simulink model "kundur_sync"  (R2023b)
settings: Solver=ode23tb  StartTime=0.0  StopTime=200  MaxStep=1/60  RelTol=1e-3
InitFcn:
  | SolarInverter_Params();
values from neighbouring files (symbols this model uses):
  Fnom = 60    [SolarInverter_Params.m]
  Pnom = 900e6    (= 900000000)    [SolarInverter_Params.m]
  reec_dbd1 = -0.1    [SolarInverter_Params.m]
  reec_dbd2 = 0.1    [SolarInverter_Params.m]
  reec_dPmax = 0.1    [SolarInverter_Params.m]
  reec_dPmin = -0.1    [SolarInverter_Params.m]
  reec_Imax = 1    [SolarInverter_Params.m]
  reec_Iqhl = 1.0    (= 1)    [SolarInverter_Params.m]
  reec_Iqll = -0.4    [SolarInverter_Params.m]
  reec_Kqi = 0.0    (= 0)    [SolarInverter_Params.m]
  reec_Kqp = 0    [SolarInverter_Params.m]
  reec_Kvi = 0.0    (= 0)    [SolarInverter_Params.m]
  reec_Kvp = 0.1    [SolarInverter_Params.m]
  reec_Pmax = 1.0    (= 1)    [SolarInverter_Params.m]
  reec_Pmin = 0    [SolarInverter_Params.m]
  reec_Qmax = 0.435    [SolarInverter_Params.m]
  reec_Qmin = -0.435    [SolarInverter_Params.m]
  reec_Tiq = 0.02    [SolarInverter_Params.m]
  reec_Tp = 0.02    [SolarInverter_Params.m]
  reec_Tpord = 0.1    [SolarInverter_Params.m]
  reec_Trv = 0.01    [SolarInverter_Params.m]
  reec_Vdip = 0.9    [SolarInverter_Params.m]
  reec_Vmax = 1.10    (= 1.1)    [SolarInverter_Params.m]
  reec_Vmin = 0.9    [SolarInverter_Params.m]
  reec_Vup = 1.15    [SolarInverter_Params.m]
  regc_Brkpt = 0.9    [SolarInverter_Params.m]
  regc_Iolim = -1.2    [SolarInverter_Params.m]
  regc_Iqrmax = 999.9    [SolarInverter_Params.m]
  regc_Iqrmin = -999.9    [SolarInverter_Params.m]
  regc_Ivpnt0 = 0.4    [SolarInverter_Params.m]
  regc_Ivpnt1 = 0.8    [SolarInverter_Params.m]
  regc_Khv = 0.0    (= 0)    [SolarInverter_Params.m]
  regc_Lvpl1 = 1.0    (= 1)    [SolarInverter_Params.m]
  regc_Lvplsw = 0    [SolarInverter_Params.m]
  regc_rrpwr = 10    [SolarInverter_Params.m]
  regc_Tfltr = 0.02    [SolarInverter_Params.m]
  regc_Tg = 0.1    [SolarInverter_Params.m]
  regc_Volim = 1.1    [SolarInverter_Params.m]
  regc_Zerox = 0.5    [SolarInverter_Params.m]
  repc_db1 = 0    [SolarInverter_Params.m]
  repc_Ddn = 20    [SolarInverter_Params.m]
  repc_Dup = 0    [SolarInverter_Params.m]
  repc_emax = 999    [SolarInverter_Params.m]
  repc_emin = -999    [SolarInverter_Params.m]
  repc_fdbd1 = 0.01*0    (= 0)    [SolarInverter_Params.m]
  repc_fdbd2 = -0.01*0    (= 0)    [SolarInverter_Params.m]
  repc_femax = 999    [SolarInverter_Params.m]
  repc_femin = -999    [SolarInverter_Params.m]
  repc_Kc = 0.05    [SolarInverter_Params.m]
  repc_Ki = 1.8    [SolarInverter_Params.m]
  repc_Kig = 0.5    [SolarInverter_Params.m]
  repc_Kp = 0.6    [SolarInverter_Params.m]
  repc_Kpg = 0.1    [SolarInverter_Params.m]
  repc_Pmax = 1    [SolarInverter_Params.m]
  repc_Pmin = 0    [SolarInverter_Params.m]
  repc_Qmax = 0.435    [SolarInverter_Params.m]
  repc_Qmin = -0.435    [SolarInverter_Params.m]
  repc_Rc = 0    [SolarInverter_Params.m]
  repc_Tfltr = 0.02    [SolarInverter_Params.m]
  repc_Tft = 0.5    [SolarInverter_Params.m]
  repc_Tfv = 0.8    [SolarInverter_Params.m]
  repc_Tlag = 0.2    [SolarInverter_Params.m]
  repc_Tp = 0.25    [SolarInverter_Params.m]
  repc_Vfrz = 0.7    [SolarInverter_Params.m]
  repc_Xc = 0    [SolarInverter_Params.m]
  Vnom = 230e3    (= 230000)    [SolarInverter_Params.m]
undefined symbols (not defined in the file or in its folder): D1, Delta, gcbh, j, k_fault, k_pulse, sps_rtmsupport
libraries: powerlib_extras x24, simulink x13, spsLoadFlowBusLib x12, spsThreePhaseVIMeasurementLib x11, spsThreePhasePISectionLineLib x8, spsThreePhaseTransformerTwoWindingsLib x5, spsThreePhaseParallelRLCLoadLib x4, spsSynchronousMachinepuStandardLib x4, spsExcitationSystemLib x4, spsSteamTurbineandGovernorLib x4, spsGenericPowerSystemStabilizerLib x4, spsControlledCurrentSourceLib x2
(part 2 of 3)

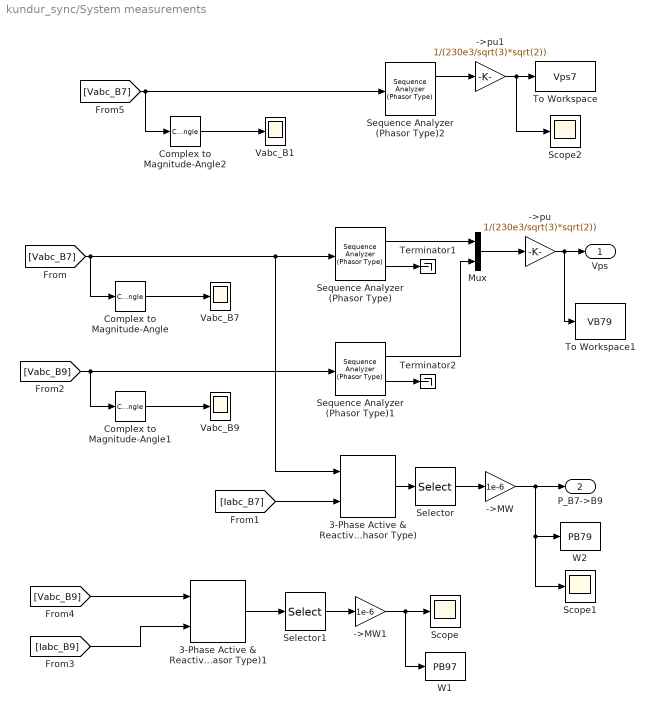
== system kundur_sync/System measurements ==
  ->MW : Gain  Gain=1e-6  SaturateOnIntegerOverflow=on  OutDataTypeStr=Inherit: Same as input  ParamDataTypeStr=Inherit: Same as input
  ->MW1 : Gain  Gain=1e-6  SaturateOnIntegerOverflow=on  OutDataTypeStr=Inherit: Same as input  ParamDataTypeStr=Inherit: Same as input
  ->pu : Gain  Gain=1/(230e3/sqrt(3)*sqrt(2))  SaturateOnIntegerOverflow=on  OutDataTypeStr=Inherit: Same as input  ParamDataTypeStr=Inherit: Same as input
  ->pu1 : Gain  Gain=1/(230e3/sqrt(3)*sqrt(2))  SaturateOnIntegerOverflow=on  OutDataTypeStr=Inherit: Same as input  ParamDataTypeStr=Inherit: Same as input
  3-Phase Active & Reactive Power (Phasor Type) : powerlib_extras/Phasor Library/3-Phase Active & Reactive Power (Phasor Type)
  3-Phase Active & Reactive Power (Phasor Type)1 : powerlib_extras/Phasor Library/3-Phase Active & Reactive Power (Phasor Type)
  Complex to Magnitude-Angle : ComplexToMagnitudeAngle  Output=Magnitude
  Complex to Magnitude-Angle1 : ComplexToMagnitudeAngle  Output=Magnitude
  Complex to Magnitude-Angle2 : ComplexToMagnitudeAngle  Output=Magnitude
  Mux : Mux  Inputs=2
  Scope : Scope
  Scope1 : Scope
  Scope2 : Scope
  Selector : Selector  InputPortWidth=2  IndexOptions=Index vector (dialog)  Indices=1  OutputSizes=1
  Selector1 : Selector  InputPortWidth=2  IndexOptions=Index vector (dialog)  Indices=1  OutputSizes=1
  Sequence Analyzer (Phasor Type) : powerlib_extras/Phasor Library/Sequence Analyzer (Phasor Type)  seq=Positive
  Sequence Analyzer (Phasor Type)1 : powerlib_extras/Phasor Library/Sequence Analyzer (Phasor Type)  seq=Positive
  Sequence Analyzer (Phasor Type)2 : powerlib_extras/Phasor Library/Sequence Analyzer (Phasor Type)  seq=Positive
  Terminator1 : Terminator
  Terminator2 : Terminator
  To Workspace : ToWorkspace  VariableName=Vps7  SampleTime=1/60
  To Workspace1 : ToWorkspace  VariableName=VB79  SampleTime=1/60
  Vabc_B1 : Scope
  Vabc_B7 : Scope
  Vabc_B9 : Scope
  W1 : ToWorkspace  VariableName=PB97  SampleTime=1/60
  W2 : ToWorkspace  VariableName=PB79  SampleTime=1/60
  Vps : Outport  VectorParamsAs1DForOutWhenUnconnected=off
  P_B7->B9 : Outport  Port=2  VectorParamsAs1DForOutWhenUnconnected=off
  wires:
  Mux/1 -> ->pu/1
  ->MW/1 -> P_B7->B9/1, Scope1/1, W2/1
  Complex to Magnitude-Angle/1 -> Vabc_B7/1
  Sequence Analyzer (Phasor Type)/1 -> Mux/1
  Selector/1 -> ->MW/1
  Sequence Analyzer (Phasor Type)/2 -> Terminator1/1
  ->pu/1 -> To Workspace1/1, Vps/1
  [Iabc_B9] -> 3-Phase Active & Reactive Power (Phasor Type)1/2
  [Iabc_B7] -> 3-Phase Active & Reactive Power (Phasor Type)/2
  3-Phase Active & Reactive Power (Phasor Type)/1 -> Selector/1
  Sequence Analyzer (Phasor Type)1/1 -> Mux/2
  Complex to Magnitude-Angle1/1 -> Vabc_B9/1
  [Vabc_B9] -> Sequence Analyzer (Phasor Type)1/1, Complex to Magnitude-Angle1/1
  [Vabc_B7] -> Sequence Analyzer (Phasor Type)/1, 3-Phase Active & Reactive Power (Phasor Type)/1, Complex to Magnitude-Angle/1
  Sequence Analyzer (Phasor Type)1/2 -> Terminator2/1
  [Vabc_B9] -> 3-Phase Active & Reactive Power (Phasor Type)1/1
  ->MW1/1 -> Scope/1, W1/1
  3-Phase Active & Reactive Power (Phasor Type)1/1 -> Selector1/1
  Selector1/1 -> ->MW1/1
  Complex to Magnitude-Angle2/1 -> Vabc_B1/1
  [Vabc_B7] -> Sequence Analyzer (Phasor Type)2/1, Complex to Magnitude-Angle2/1
  Sequence Analyzer (Phasor Type)2/1 -> ->pu1/1
  ->pu1/1 -> Scope2/1, To Workspace/1

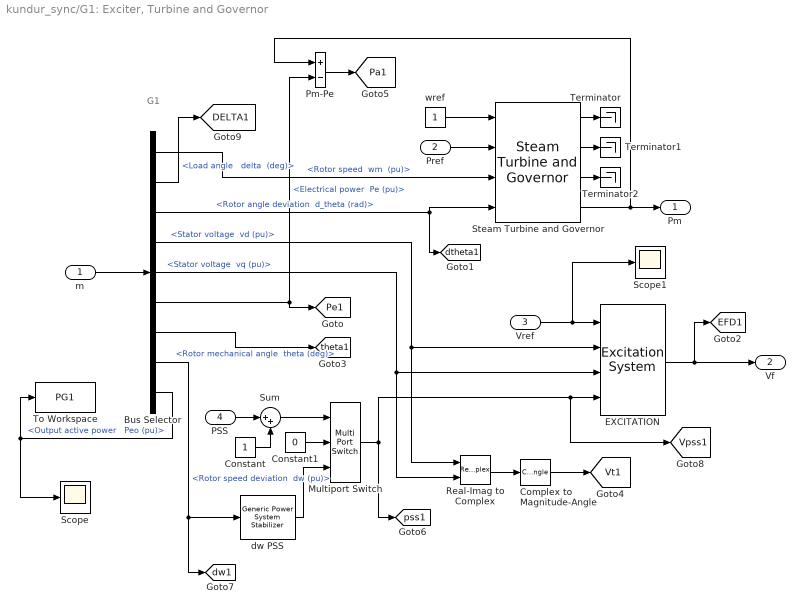
== system kundur_sync/G1: Exciter, Turbine and Governor ==
  note: G1
  m : Inport
  Pref : Inport  Port=2
  Vref : Inport  Port=3
  PSS : Inport  Port=4
  Bus Selector : BusSelector  OutputSignals="Mechanical.Rotor speed  wm  (pu),Load angle   delta  (deg),Mechanical.Rotor angle deviation  d_theta (rad),dq0 components.Stator voltage  vd (pu),dq0 components.Stator voltage  vq (pu),Mechanical.Electrical power  Pe (pu),Mechanical.Rotor mechanical angle  theta (deg),Mechanical.Rotor speed deviation  dw (pu),Output active power   Peo (pu)"
  Complex to Magnitude-Angle : ComplexToMagnitudeAngle  Output=Magnitude
  Constant : Constant
  Constant1 : Constant  Value=0
  EXCITATION : spsExcitationSystemLib/Excitation System  tr=20e-3  reg=[ 200, 0.001 ]  exc=[ 1, 0 ]  tgr=[ 0, 0 ]  damp=[ 0, 0 ]  sat=[ 0, 0 ]  lim=[ 0 , 12.3, 0 ]  v0=[1.03 1.9356]
  Multiport Switch : MultiPortSwitch  Inputs=2  SaturateOnIntegerOverflow=off  InputSameDT=off
  Pm-Pe : Sum  Inputs=+-
  Real-Imag to Complex : RealImagToComplex
  Scope : Scope
  Scope1 : Scope
  Sum : Sum  Inputs=|++
  Terminator : Terminator
  Terminator1 : Terminator
  Terminator2 : Terminator
  To Workspace : ToWorkspace  VariableName=PG1  SampleTime=1/60
  Steam Turbine and Governor : spsSteamTurbineandGovernorLib/Steam Turbine and Governor  gentype=Tandem-compound (single mass)  reg1="[ 1  0.05    0 ]"  reg2="[ 0.001  0.15 ]"  reg3="[ -0.1  0.1  0  4.496]"  N=3600  turb1="[ 0  10  3.3  0.5 ]"  turb2="[ 0   0.36   0.36  0.28 ]"  HA="[  1.5498   0.24894  0  0 ]"  KA="[  83.47  42.702  0  0 ]"  DA="[  0.3104  0.05  0  0 ]*8"  ini1=0.7793  ini2=[2.7247e-008,-120.13]
      settings: LibrarySourceBlock=|
      | sps_lib/Electrical Machines/Synchronous Machine Control/Steam Turbine
      | and Governor
  dw PSS : spsGenericPowerSystemStabilizerLib/Generic Power System Stabilizer  Tsensor=15e-3  K=30  Twashout=10  Tleadlag1=[50e-3 20e-3]  Tleadlag2=[3 5.4]  VSlimits=[-0.15 0.15]  Vinit=0  Plot_On=off  MagdB_On=on  FreqRange=logspace(-2,2,500)
      settings: LibrarySourceBlock=|
      | sps_lib/Electrical Machines/Synchronous Machine Control/Generic
      | Power System Stabilizer
  wref : Constant
  Pm : Outport  VectorParamsAs1DForOutWhenUnconnected=off
  Vf : Outport  Port=2  VectorParamsAs1DForOutWhenUnconnected=off
  tag scope: DELTA1=global, EFD1=global, Pa1=global, Pe1=global, Vpss1=global, Vt1=global, dtheta1=global, dw1=global, pss1=global, theta1=global
  wires:
  m/1 -> Bus Selector/1
  Steam Turbine and Governor/4 -> Pm/1, Pm-Pe/1
  Bus Selector/1 -> Steam Turbine and Governor/3  "<Rotor speed  wm  (pu)>"
  Bus Selector/3 -> Steam Turbine and Governor/4, [dtheta1]  "<Rotor angle deviation  d_theta (rad)>"
  Bus Selector/4 -> Real-Imag to Complex/1, EXCITATION/2  "<Stator voltage  vd (pu)>"
  Bus Selector/5 -> Real-Imag to Complex/2, EXCITATION/3  "<Stator voltage  vq (pu)>"
  wref/1 -> Steam Turbine and Governor/1
  Pref/1 -> Steam Turbine and Governor/2
  Steam Turbine and Governor/1 -> Terminator/1
  Steam Turbine and Governor/2 -> Terminator1/1
  Steam Turbine and Governor/3 -> Terminator2/1
  Bus Selector/6 -> Pm-Pe/2, [Pe1]  "<Electrical power  Pe (pu)>"
  Bus Selector/7 -> [theta1]  "<Rotor mechanical angle  theta (deg)>"
  Real-Imag to Complex/1 -> Complex to Magnitude-Angle/1
  Complex to Magnitude-Angle/1 -> [Vt1]
  Bus Selector/8 -> [dw1], dw PSS/1  "<Rotor speed deviation  dw (pu)>"
  Sum/1 -> Multiport Switch/1
  PSS/1 -> Sum/1
  Constant/1 -> Sum/2
  Constant1/1 -> Multiport Switch/2
  dw PSS/1 -> Multiport Switch/3
  Multiport Switch/1 -> [Vpss1], EXCITATION/4, [pss1]
  Pm-Pe/1 -> [Pa1]
  Bus Selector/9 -> Scope/1, To Workspace/1  "<Output active power   Peo (pu)>"
  EXCITATION/1 -> [EFD1], Vf/1
  Vref/1 -> Scope1/1, EXCITATION/1
  Bus Selector/2 -> [DELTA1]  "<Load angle   delta  (deg)>"

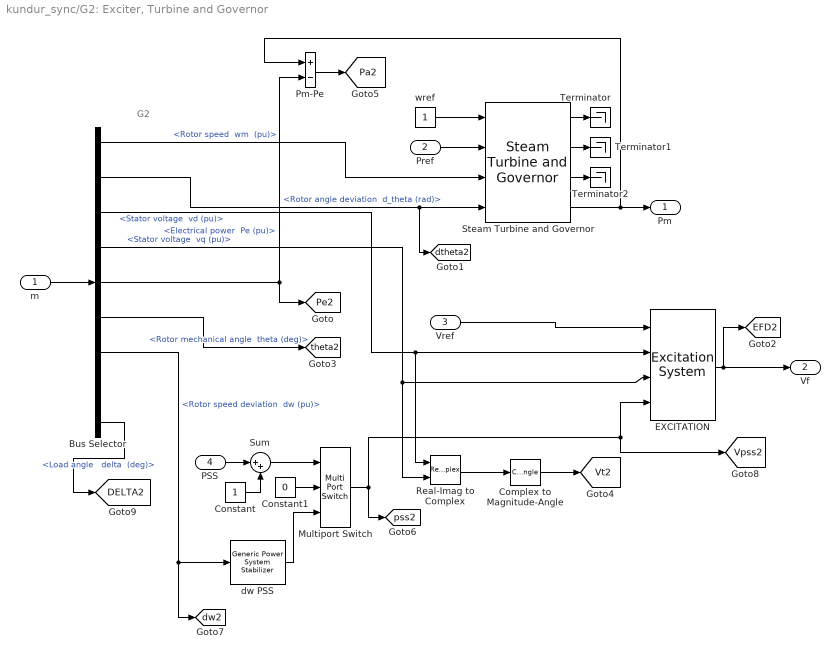
== system kundur_sync/G2: Exciter, Turbine and Governor ==
  note: G2
  m : Inport
  Pref : Inport  Port=2
  Vref : Inport  Port=3
  PSS : Inport  Port=4
  Bus Selector : BusSelector  OutputSignals="Mechanical.Rotor speed  wm  (pu),Mechanical.Rotor angle deviation  d_theta (rad),dq0 components.Stator voltage  vd (pu),dq0 components.Stator voltage  vq (pu),Mechanical.Electrical power  Pe (pu),Mechanical.Rotor mechanical angle  theta (deg),Mechanical.Rotor speed deviation  dw (pu),dq0 components.Field current  ifd (pu),Load angle   delta  (deg)"
  Complex to Magnitude-Angle : ComplexToMagnitudeAngle  Output=Magnitude
  Constant : Constant
  Constant1 : Constant  Value=0
  EXCITATION : spsExcitationSystemLib/Excitation System  tr=20e-3  reg=[ 200, 0.001 ]  exc=[ 1, 0 ]  tgr=[ 0, 0 ]  damp=[ 0, 0 ]  sat=[ 0, 0 ]  lim=[ 0 , 12.3, 0 ]  v0=[1.01 2.0029]
  Multiport Switch : MultiPortSwitch  Inputs=2  SaturateOnIntegerOverflow=off  InputSameDT=off
  Pm-Pe : Sum  Inputs=+-
  Real-Imag to Complex : RealImagToComplex
  Sum : Sum  Inputs=|++
  Terminator : Terminator
  Terminator1 : Terminator
  Terminator2 : Terminator
  Steam Turbine and Governor : spsSteamTurbineandGovernorLib/Steam Turbine and Governor  gentype=Tandem-compound (single mass)  reg1="[ 1  0.05    0 ]"  reg2="[ 0.001  0.15 ]"  reg3="[ -0.1  0.1  0  4.496]"  N=3600  turb1="[ 0  10   3.3   0.5   ]"  turb2="[ 0   0.36   0.36  0.28 ]"  HA="[  1.5498   0.24894  0  0 ]"  KA="[  83.47  42.702  0  0 ]"  DA="[  0.3104  0.05  0  0 ]*8"  ini1=0.77941  ini2=[2.7247e-008,-120.13]
      settings: LibrarySourceBlock=|
      | sps_lib/Electrical Machines/Synchronous Machine Control/Steam Turbine
      | and Governor
  dw PSS : spsGenericPowerSystemStabilizerLib/Generic Power System Stabilizer  Tsensor=15e-3  K=30  Twashout=10  Tleadlag1=[50e-3 20e-3]  Tleadlag2=[3 5.4]  VSlimits=[-0.15 0.15]  Vinit=0  Plot_On=off  MagdB_On=on  FreqRange=logspace(-2,2,500)
      settings: LibrarySourceBlock=|
      | sps_lib/Electrical Machines/Synchronous Machine Control/Generic
      | Power System Stabilizer
  wref : Constant
  Pm : Outport  VectorParamsAs1DForOutWhenUnconnected=off
  Vf : Outport  Port=2  VectorParamsAs1DForOutWhenUnconnected=off
  tag scope: DELTA2=global, EFD2=global, Pa2=global, Pe2=global, Vpss2=global, Vt2=global, dtheta2=global, dw2=global, pss2=global, theta2=global
  wires:
  m/1 -> Bus Selector/1
  EXCITATION/1 -> Vf/1, [EFD2]
  Steam Turbine and Governor/4 -> Pm/1, Pm-Pe/1
  Bus Selector/1 -> Steam Turbine and Governor/3  "<Rotor speed  wm  (pu)>"
  Bus Selector/2 -> Steam Turbine and Governor/4, [dtheta2]  "<Rotor angle deviation  d_theta (rad)>"
  Bus Selector/3 -> Real-Imag to Complex/1, EXCITATION/2  "<Stator voltage  vd (pu)>"
  Bus Selector/4 -> EXCITATION/3, Real-Imag to Complex/2  "<Stator voltage  vq (pu)>"
  wref/1 -> Steam Turbine and Governor/1
  Pref/1 -> Steam Turbine and Governor/2
  Steam Turbine and Governor/1 -> Terminator/1
  Steam Turbine and Governor/2 -> Terminator1/1
  Steam Turbine and Governor/3 -> Terminator2/1
  Vref/1 -> EXCITATION/1
  Bus Selector/5 -> [Pe2], Pm-Pe/2  "<Electrical power  Pe (pu)>"
  Bus Selector/6 -> [theta2]  "<Rotor mechanical angle  theta (deg)>"
  Real-Imag to Complex/1 -> Complex to Magnitude-Angle/1
  Complex to Magnitude-Angle/1 -> [Vt2]
  Sum/1 -> Multiport Switch/1
  PSS/1 -> Sum/1
  Constant/1 -> Sum/2
  Constant1/1 -> Multiport Switch/2
  dw PSS/1 -> Multiport Switch/3
  Multiport Switch/1 -> [Vpss2], EXCITATION/4, [pss2]
  Pm-Pe/1 -> [Pa2]
  Bus Selector/7 -> [dw2], dw PSS/1  "<Rotor speed deviation  dw (pu)>"
  Bus Selector/9 -> [DELTA2]  "<Load angle   delta  (deg)>"

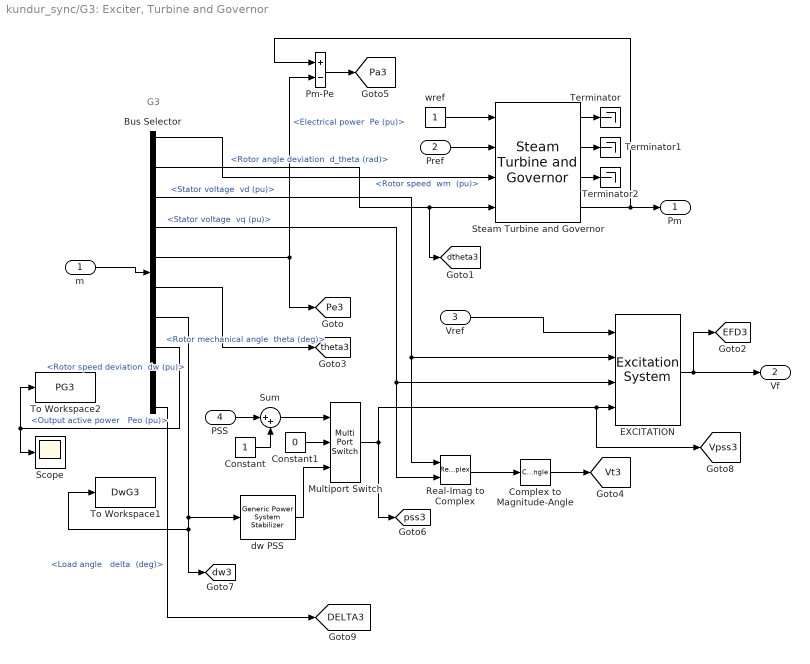
== system kundur_sync/G3: Exciter, Turbine and Governor ==
  note: G3
  m : Inport
  Pref : Inport  Port=2
  Vref : Inport  Port=3
  PSS : Inport  Port=4
  Bus Selector : BusSelector  OutputSignals="Mechanical.Rotor speed  wm  (pu),Mechanical.Rotor angle deviation  d_theta (rad),dq0 components.Stator voltage  vd (pu),dq0 components.Stator voltage  vq (pu),Mechanical.Electrical power  Pe (pu),Mechanical.Rotor mechanical angle  theta (deg),Mechanical.Rotor speed deviation  dw (pu),Output active power   Peo (pu),dq0 components.Field current  ifd (pu),Load angle   delta  (deg)"
  Complex to Magnitude-Angle : ComplexToMagnitudeAngle  Output=Magnitude
  Constant : Constant
  Constant1 : Constant  Value=0
  EXCITATION : spsExcitationSystemLib/Excitation System  tr=20e-3  reg=[ 200, 0.001 ]  exc=[ 1, 0 ]  tgr=[ 0, 0 ]  damp=[ 0, 0 ]  sat=[ 0, 0 ]  lim=[ 0 , 12.3, 0 ]  v0=[1.03 1.9474]
  Multiport Switch : MultiPortSwitch  Inputs=2  SaturateOnIntegerOverflow=off  InputSameDT=off
  Pm-Pe : Sum  Inputs=+-
  Real-Imag to Complex : RealImagToComplex
  Scope : Scope
  Sum : Sum  Inputs=|++
  Terminator : Terminator
  Terminator1 : Terminator
  Terminator2 : Terminator
  To Workspace1 : ToWorkspace  VariableName=DwG3  SampleTime=1/60
  To Workspace2 : ToWorkspace  VariableName=PG3  SampleTime=1/60
  Steam Turbine and Governor : spsSteamTurbineandGovernorLib/Steam Turbine and Governor  gentype=Tandem-compound (single mass)  reg1="[ 1  0.05    0 ]"  reg2="[ 0.001  0.15 ]"  reg3="[ -0.1  0.1  0  4.496]"  N=3600  turb1="[ 0  10   3.3   0.5   ]"  turb2="[ 0   0.36   0.36  0.28 ]"  HA="[  1.5498   0.24894  0  0 ]"  KA="[  83.47  42.702  0  0 ]"  DA="[  0.3104  0.05  0  0 ]*8"  ini1=0.80012  ini2=[2.7247e-008,-120.13]
      settings: LibrarySourceBlock=|
      | sps_lib/Electrical Machines/Synchronous Machine Control/Steam Turbine
      | and Governor
  dw PSS : spsGenericPowerSystemStabilizerLib/Generic Power System Stabilizer  Tsensor=15e-3  K=30  Twashout=10  Tleadlag1=[50e-3 20e-3]  Tleadlag2=[3 5.4]  VSlimits=[-0.15 0.15]  Vinit=0  Plot_On=off  MagdB_On=on  FreqRange=logspace(-2,2,500)
      settings: LibrarySourceBlock=|
      | sps_lib/Electrical Machines/Synchronous Machine Control/Generic
      | Power System Stabilizer
  wref : Constant
  Pm : Outport  VectorParamsAs1DForOutWhenUnconnected=off
  Vf : Outport  Port=2  VectorParamsAs1DForOutWhenUnconnected=off
  tag scope: DELTA3=global, EFD3=global, Pa3=global, Pe3=global, Vpss3=global, Vt3=global, dtheta3=global, dw3=global, pss3=global, theta3=global
  wires:
  m/1 -> Bus Selector/1
  EXCITATION/1 -> Vf/1, [EFD3]
  Steam Turbine and Governor/4 -> Pm/1, Pm-Pe/1
  Bus Selector/1 -> Steam Turbine and Governor/3  "<Rotor speed  wm  (pu)>"
  Bus Selector/2 -> Steam Turbine and Governor/4, [dtheta3]  "<Rotor angle deviation  d_theta (rad)>"
  Bus Selector/3 -> EXCITATION/2, Real-Imag to Complex/1  "<Stator voltage  vd (pu)>"
  Bus Selector/4 -> Real-Imag to Complex/2, EXCITATION/3  "<Stator voltage  vq (pu)>"
  wref/1 -> Steam Turbine and Governor/1
  Pref/1 -> Steam Turbine and Governor/2
  Steam Turbine and Governor/1 -> Terminator/1
  Steam Turbine and Governor/2 -> Terminator1/1
  Steam Turbine and Governor/3 -> Terminator2/1
  Vref/1 -> EXCITATION/1
  Bus Selector/5 -> [Pe3], Pm-Pe/2  "<Electrical power  Pe (pu)>"
  Bus Selector/6 -> [theta3]  "<Rotor mechanical angle  theta (deg)>"
  Real-Imag to Complex/1 -> Complex to Magnitude-Angle/1
  Complex to Magnitude-Angle/1 -> [Vt3]
  Sum/1 -> Multiport Switch/1
  PSS/1 -> Sum/1
  Constant/1 -> Sum/2
  Constant1/1 -> Multiport Switch/2
  dw PSS/1 -> Multiport Switch/3
  Multiport Switch/1 -> [Vpss3], EXCITATION/4, [pss3]
  Pm-Pe/1 -> [Pa3]
  Bus Selector/7 -> To Workspace1/1, [dw3], dw PSS/1  "<Rotor speed deviation  dw (pu)>"
  Bus Selector/8 -> Scope/1, To Workspace2/1  "<Output active power   Peo (pu)>"
  Bus Selector/10 -> [DELTA3]  "<Load angle   delta  (deg)>"

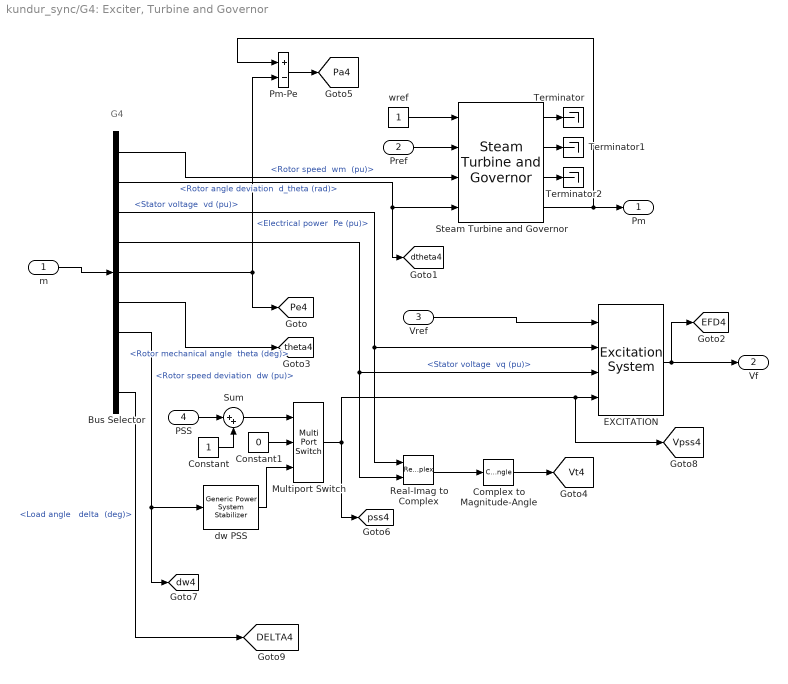
== system kundur_sync/G4: Exciter, Turbine and Governor ==
  note: G4
  m : Inport
  Pref : Inport  Port=2
  Vref : Inport  Port=3
  PSS : Inport  Port=4
  Bus Selector : BusSelector  OutputSignals="Mechanical.Rotor speed  wm  (pu),Mechanical.Rotor angle deviation  d_theta (rad),dq0 components.Stator voltage  vd (pu),dq0 components.Stator voltage  vq (pu),Mechanical.Electrical power  Pe (pu),Mechanical.Rotor mechanical angle  theta (deg),Mechanical.Rotor speed deviation  dw (pu),dq0 components.Field current  ifd (pu),Load angle   delta  (deg)"
  Complex to Magnitude-Angle : ComplexToMagnitudeAngle  Output=Magnitude
  Constant : Constant
  Constant1 : Constant  Value=0
  EXCITATION : spsExcitationSystemLib/Excitation System  tr=20e-3  reg=[ 200, 0.001 ]  exc=[ 1, 0 ]  tgr=[ 0, 0 ]  damp=[ 0, 0 ]  sat=[ 0, 0 ]  lim=[ 0 , 12.3, 0 ]  v0=[1.01 1.9533]
  Multiport Switch : MultiPortSwitch  Inputs=2  SaturateOnIntegerOverflow=off  InputSameDT=off
  Pm-Pe : Sum  Inputs=+-
  Real-Imag to Complex : RealImagToComplex
  Sum : Sum  Inputs=|++
  Terminator : Terminator
  Terminator1 : Terminator
  Terminator2 : Terminator
  Steam Turbine and Governor : spsSteamTurbineandGovernorLib/Steam Turbine and Governor  gentype=Tandem-compound (single mass)  reg1="[ 1  0.05    0 ]"  reg2="[ 0.001  0.15 ]"  reg3="[ -0.1  0.1  0  4.496]"  N=3600  turb1="[ 0  10   3.3   0.5   ]"  turb2="[ 0   0.36   0.36  0.28 ]"  HA="[  1.5498   0.24894  0  0 ]"  KA="[  83.47  42.702  0  0 ]"  DA="[  0.3104  0.05  0  0 ]*8"  ini1=0.77936  ini2=[2.7247e-008,-120.13]
      settings: LibrarySourceBlock=|
      | sps_lib/Electrical Machines/Synchronous Machine Control/Steam Turbine
      | and Governor
  dw PSS : spsGenericPowerSystemStabilizerLib/Generic Power System Stabilizer  Tsensor=15e-3  K=30  Twashout=10  Tleadlag1=[50e-3 20e-3]  Tleadlag2=[3 5.4]  VSlimits=[-0.15 0.15]  Vinit=0  Plot_On=off  MagdB_On=on  FreqRange=logspace(-2,2,500)
      settings: LibrarySourceBlock=|
      | sps_lib/Electrical Machines/Synchronous Machine Control/Generic
      | Power System Stabilizer
  wref : Constant
  Pm : Outport  VectorParamsAs1DForOutWhenUnconnected=off
  Vf : Outport  Port=2  VectorParamsAs1DForOutWhenUnconnected=off
  tag scope: DELTA4=global, EFD4=global, Pa4=global, Pe4=global, Vpss4=global, Vt4=global, dtheta4=global, dw4=global, pss4=global, theta4=global
  wires:
  m/1 -> Bus Selector/1
  EXCITATION/1 -> [EFD4], Vf/1
  Steam Turbine and Governor/4 -> Pm/1, Pm-Pe/1
  Bus Selector/1 -> Steam Turbine and Governor/3  "<Rotor speed  wm  (pu)>"
  Bus Selector/2 -> Steam Turbine and Governor/4, [dtheta4]  "<Rotor angle deviation  d_theta (rad)>"
  Bus Selector/3 -> EXCITATION/2, Real-Imag to Complex/1  "<Stator voltage  vd (pu)>"
  Bus Selector/4 -> EXCITATION/3, Real-Imag to Complex/2  "<Stator voltage  vq (pu)>"
  wref/1 -> Steam Turbine and Governor/1
  Pref/1 -> Steam Turbine and Governor/2
  Steam Turbine and Governor/1 -> Terminator/1
  Steam Turbine and Governor/2 -> Terminator1/1
  Steam Turbine and Governor/3 -> Terminator2/1
  Vref/1 -> EXCITATION/1
  Bus Selector/5 -> [Pe4], Pm-Pe/2  "<Electrical power  Pe (pu)>"
  Bus Selector/6 -> [theta4]  "<Rotor mechanical angle  theta (deg)>"
  Real-Imag to Complex/1 -> Complex to Magnitude-Angle/1
  Complex to Magnitude-Angle/1 -> [Vt4]
  Sum/1 -> Multiport Switch/1
  PSS/1 -> Sum/1
  Constant/1 -> Sum/2
  Constant1/1 -> Multiport Switch/2
  dw PSS/1 -> Multiport Switch/3
  Multiport Switch/1 -> [Vpss4], EXCITATION/4, [pss4]
  Pm-Pe/1 -> [Pa4]
  Bus Selector/7 -> [dw4], dw PSS/1  "<Rotor speed deviation  dw (pu)>"
  Bus Selector/9 -> [DELTA4]  "<Load angle   delta  (deg)>"

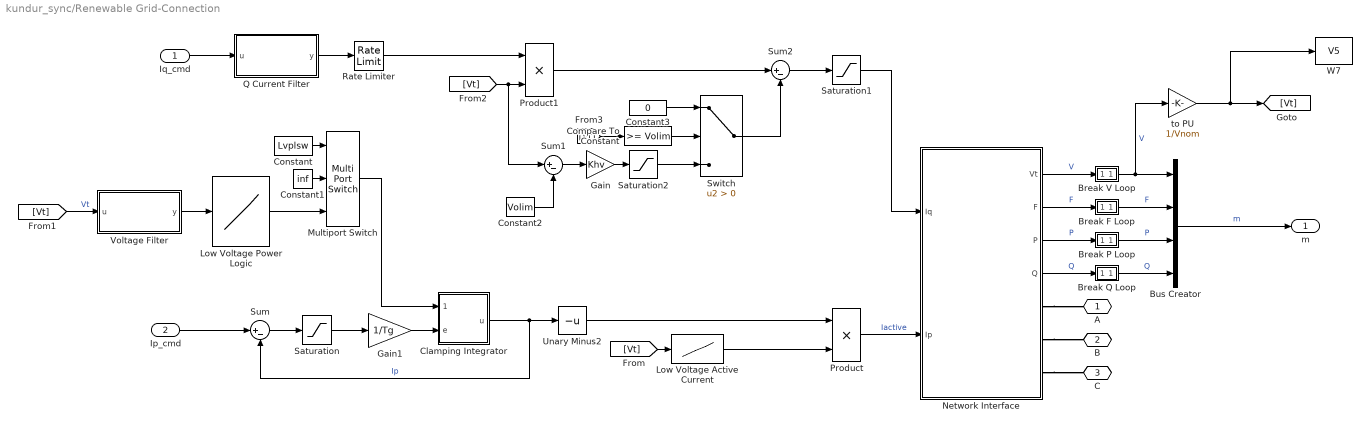
== system kundur_sync/Renewable Grid-Connection ==
  Iq_cmd : Inport
  Ip_cmd : Inport  Port=2
  Break F Loop : Subsystem  mask{tau=0.001, toPU=Fnom}
      mask prompts: toPU "Convert to PU"
  Break P Loop : Subsystem  mask{tau=0.001, toPU=Pnom}
      mask prompts: toPU "Convert to PU"
  Break Q Loop : Subsystem  mask{tau=0.001, toPU=Pnom}
      mask prompts: toPU "Convert to PU"
  Break V Loop : Subsystem  mask{tau=0.001, toPU=Vnom}
      mask prompts: toPU "Convert to PU"
  Bus Creator : BusCreator  Inputs=4
  Clamping Integrator : Subsystem
  Compare To Constant : simulink/Logic and Bit Operations/Compare To Constant  relop=>=  const=Volim  OutDataTypeStr=boolean
  Constant : Constant  Value=Lvplsw
  Constant1 : Constant  Value=inf
  Constant2 : Constant  Value=Volim
  Constant3 : Constant  Value=0
  Gain : Gain  Gain=Khv
  Gain1 : Gain  Gain=1/Tg
  Low Voltage Active Current : Lookup_n-D  NumberOfTableDimensions=1  BreakpointsForDimension1=[0 Ivpnt0 Ivpnt1 Ivpnt1*1.5]  Table=[0 0 1 1]  InternalRulePriority=Speed  RndMeth=Simplest
  Low Voltage Power Logic : Lookup_n-D  NumberOfTableDimensions=1  BreakpointsForDimension1=[0 Zerox Brkpt Brkpt*1.01 Brkpt*1.5]  Table=[0 0 Lvpl1 Lvpl1*5 Lvpl1*5]  InternalRulePriority=Speed  RndMeth=Simplest
  Multiport Switch : MultiPortSwitch  DataPortOrder=Zero-based contiguous  Inputs=2  zeroidx=on  SaturateOnIntegerOverflow=off  InputSameDT=off
  Network Interface : Subsystem
  Product : Product
  Product1 : Product
  Q Current Filter : Subsystem  mask{k=1, tau=Tg, vmax=Iqrmax, vmin=Iqrmin}
      mask Display: fprintf('1\n------------\n(1 + s Tg)');
  Rate Limiter : RateLimiter  RisingSlewLimit=Iqrmax  FallingSlewLimit=Iqrmin  SampleTimeMode=inherited
  Saturation : Saturate  UpperLimit=rrpwr  LowerLimit=-inf
  Saturation1 : Saturate  UpperLimit=inf  LowerLimit=Iolim
  Saturation2 : Saturate  UpperLimit=inf  LowerLimit=0
  Sum : Sum  Inputs=|+-
  Sum1 : Sum  Inputs=|+-
  Sum2 : Sum  Inputs=|+-
  Switch : Switch  Criteria=u2 > Threshold  SaturateOnIntegerOverflow=off  InputSameDT=off
  Unary Minus2 : UnaryMinus
  Voltage Filter : Subsystem  mask{k=1, tau=Tfltr, vmax=inf, vmin=-inf}
      mask Display: fprintf('1\n------------\n(1 + s Tfltr)');
  W7 : ToWorkspace  VariableName=V5  SampleTime=1/60
  to PU : Gain  Gain=1/Vnom
  A : PMIOPort  Side=Right
  B : PMIOPort  Port=2  Side=Right
  C : PMIOPort  Port=3  Side=Right
  m : Outport  VectorParamsAs1DForOutWhenUnconnected=off
  wires:
  [Vt] -> Voltage Filter/1(u)  "Vt"
  Q Current Filter/1(y) -> Rate Limiter/1
  Network Interface/4(Q) -> Break Q Loop/1(u)  "Q"
  Constant3/1 -> Switch/1
  Network Interface/1(Vt) -> Break V Loop/1(u)  "V"
  Iq_cmd/1 -> Q Current Filter/1(u)
  Gain/1 -> Saturation2/1
  Network Interface/3(P) -> Break P Loop/1(u)  "P"
  Voltage Filter/1(y) -> Low Voltage Power Logic/1
  Constant1/1 -> Multiport Switch/2
  Sum/1 -> Saturation/1
  Constant/1 -> Multiport Switch/1
  Product/1 -> Network Interface/2(Ip)  "Iactive"
  Low Voltage Active Current/1 -> Product/2
  Multiport Switch/1 -> Clamping Integrator/1(LVMax)
  Clamping Integrator/1(u) -> Sum/2, Unary Minus2/1  "Ip"
  Gain1/1 -> Clamping Integrator/2(e)
  [Vt] -> Compare To Constant/1
  Saturation/1 -> Gain1/1
  [Vt] -> Low Voltage Active Current/1
  Constant2/1 -> Sum1/2
  Saturation1/1 -> Network Interface/1(Iq)
  Product1/1 -> Sum2/1
  Sum1/1 -> Gain/1
  Rate Limiter/1 -> Product1/1
  Saturation2/1 -> Switch/3
  [Vt] -> Sum1/1, Product1/2
  Low Voltage Power Logic/1 -> Multiport Switch/3
  Compare To Constant/1 -> Switch/2
  Switch/1 -> Sum2/2
  Bus Creator/1 -> m/1  "m"
  Sum2/1 -> Saturation1/1
  Ip_cmd/1 -> Sum/1
  Network Interface/2(F) -> Break F Loop/1(u)  "F"
  Unary Minus2/1 -> Product/1
  to PU/1 -> W7/1, [Vt]
  Break V Loop/1(y) -> to PU/1, Bus Creator/1  "V"
  Break F Loop/1(y) -> Bus Creator/2  "F"
  Break P Loop/1(y) -> Bus Creator/3  "P"
  Break Q Loop/1(y) -> Bus Creator/4  "Q"
  connections:
  Network Interface/RConn3 -- C/RConn1
  Network Interface/RConn1 -- A/RConn1
  Network Interface/RConn2 -- B/RConn1

== system kundur_sync/Selection ==
  In1 : Inport
  Bus Selector : BusSelector  OutputSignals=V,F,P,Q
  Mux : Mux  Inputs=2
  Mux1 : Mux  Inputs=2
  Mux2 : Mux  Inputs=2
  P to PU : Gain  Gain=1/Pnom
  Q to PU : Gain  Gain=1/Pnom
  V to PU : Gain  Gain=1/Vnom
  Out1 : Outport
  <F> : Outport  Port=2
  Out3 : Outport  Port=3
  Out4 : Outport  Port=4
  wires:
  Bus Selector/4 -> Q to PU/1  "<Q>"
  Bus Selector/3 -> P to PU/1  "<P>"
  V to PU/1 -> Mux2/1
  Bus Selector/1 -> V to PU/1  "<V>"
  [Vref] -> Mux2/2
  Q to PU/1 -> Mux1/1
  P to PU/1 -> Mux/1
  [Qref] -> Mux1/2
  [Pref] -> Mux/2
  Bus Selector/2 -> <F>/1  "<F>"
  Mux/1 -> Out3/1
  Mux2/1 -> Out1/1
  Mux1/1 -> Out4/1
  In1/1 -> Bus Selector/1

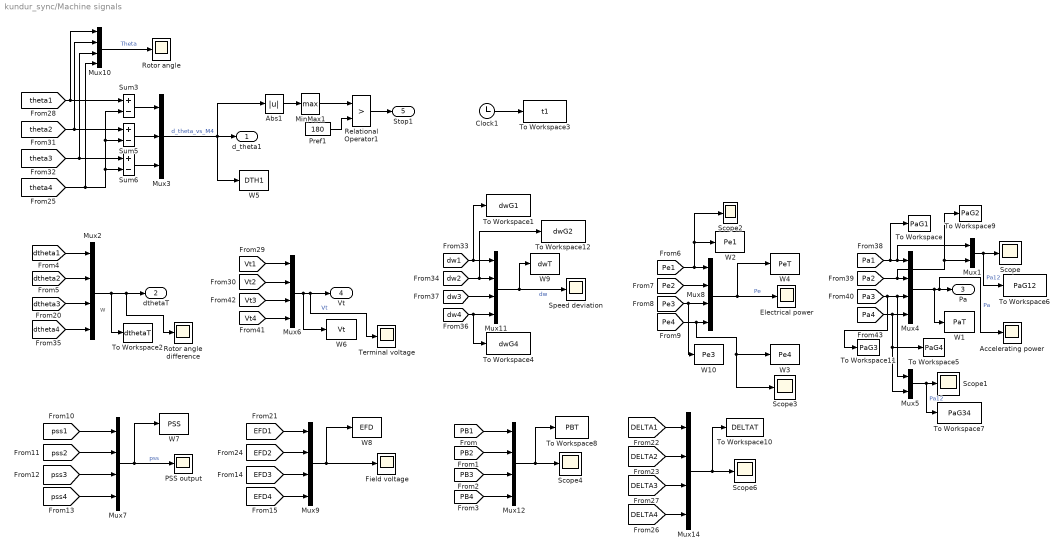
== system kundur_sync/Machine signals ==
  note: w
  Abs1 : Abs
  Clock1 : Clock
  Speed deviation : Scope
  Rotor angle difference : Scope
  MinMax1 : MinMax  Function=max  InputSameDT=on  SaturateOnIntegerOverflow=on
  Mux1 : Mux  Inputs=2
  Mux{2,4,6..12,14} (10 alike) : Mux
  Mux3 : Mux  Inputs=3
  Mux5 : Mux  Inputs=2
  Electrical power : Scope
  Accelerating power : Scope
  Pref1 : Constant  Value=180
  Relational Operator1 : RelationalOperator  Operator=>
  Scope{,1..4,6} (6 alike) : Scope
  PSS output : Scope
  Sum3 : Sum  Inputs=+-  InputSameDT=on  SaturateOnIntegerOverflow=on  OutDataTypeStr=Inherit: Same as first input
  Sum5 : Sum  Inputs=+-  InputSameDT=on  SaturateOnIntegerOverflow=on  OutDataTypeStr=Inherit: Same as first input
  Sum6 : Sum  Inputs=+-  InputSameDT=on  SaturateOnIntegerOverflow=on  OutDataTypeStr=Inherit: Same as first input
  Rotor angle : Scope
  To Workspace : ToWorkspace  VariableName=PaG1  SampleTime=1/60
  To Workspace1 : ToWorkspace  VariableName=dwG1  SampleTime=1/60
  To Workspace10 : ToWorkspace  VariableName=DELTAT  SampleTime=1/60
  To Workspace11 : ToWorkspace  VariableName=PaG3  SampleTime=1/60
  To Workspace12 : ToWorkspace  VariableName=dwG2  SampleTime=1/60
  To Workspace2 : ToWorkspace  VariableName=dthetaT  SampleTime=1/60
  To Workspace3 : ToWorkspace  VariableName=t1  SampleTime=1/60
  To Workspace4 : ToWorkspace  VariableName=dwG4  SampleTime=1/60
  To Workspace5 : ToWorkspace  VariableName=PaG4  SampleTime=1/60
  To Workspace6 : ToWorkspace  VariableName=PaG12  SampleTime=1/60
  To Workspace7 : ToWorkspace  VariableName=PaG34  SampleTime=1/60
  To Workspace8 : ToWorkspace  VariableName=PBT  SampleTime=1/60
  To Workspace9 : ToWorkspace  VariableName=PaG2  SampleTime=1/60
  Field voltage : Scope
  Terminal voltage : Scope
  W1 : ToWorkspace  VariableName=PaT  SampleTime=1/60
  W10 : ToWorkspace  VariableName=Pe3  SampleTime=1/60
  W2 : ToWorkspace  VariableName=Pe1  SampleTime=1/60
  W3 : ToWorkspace  VariableName=Pe4  SampleTime=1/60
  W4 : ToWorkspace  VariableName=PeT  SampleTime=1/60
  W5 : ToWorkspace  VariableName=DTH1  SampleTime=1/60
  W6 : ToWorkspace  VariableName=Vt  SampleTime=1/60
  W7 : ToWorkspace  VariableName=PSS  SampleTime=1/60
  W8 : ToWorkspace  VariableName=EFD  SampleTime=1/60
  W9 : ToWorkspace  VariableName=dwT  SampleTime=1/60
  d_theta1 : Outport  VectorParamsAs1DForOutWhenUnconnected=off
  dthetaT : Outport  Port=2  VectorParamsAs1DForOutWhenUnconnected=off
  Pa : Outport  Port=3  VectorParamsAs1DForOutWhenUnconnected=off
  Vt : Outport  Port=4  VectorParamsAs1DForOutWhenUnconnected=off
  Stop1 : Outport  Port=5  VectorParamsAs1DForOutWhenUnconnected=off
  wires:
  Sum3/1 -> Mux3/1
  [Pa4] -> Mux5/2, To Workspace5/1, Mux4/4
  [dw1] -> Mux11/1, To Workspace1/1
  Mux10/1 -> Rotor angle/1  "Theta"
  Mux11/1 -> Speed deviation/1, W9/1  "dw"
  MinMax1/1 -> Relational Operator1/1
  Pref1/1 -> Relational Operator1/2
  [dw2] -> To Workspace12/1, Mux11/2
  [dw3] -> Mux11/3
  [dw4] -> Mux11/4, To Workspace4/1
  [theta3] -> Mux10/3, Sum6/1
  Clock1/1 -> To Workspace3/1
  [pss4] -> Mux7/4
  Mux2/1 -> To Workspace2/1, Rotor angle difference/1, dthetaT/1
  Abs1/1 -> MinMax1/1
  Sum6/1 -> Mux3/3
  [theta1] -> Mux10/1, Sum3/1
  [Pa2] -> To Workspace9/1, Mux1/2, Mux4/2
  [Pe2] -> Mux8/2
  [Vt1] -> Mux6/1
  [Vt3] -> Mux6/3
  [dtheta3] -> Mux2/3
  [EFD3] -> Mux9/3
  [pss2] -> Mux7/2
  Mux8/1 -> Electrical power/1, W4/1  "Pe"
  [Vt2] -> Mux6/2
  [theta4] -> Mux10/4, Sum6/2, Sum5/2, Sum3/2
  Relational Operator1/1 -> Stop1/1
  [EFD4] -> Mux9/4
  Mux3/1 -> d_theta1/1, Abs1/1, W5/1  "d_theta_vs_M4"
  Mux7/1 -> PSS output/1, W7/1  "pss"
  [theta2] -> Mux10/2, Sum5/1
  Sum5/1 -> Mux3/2
  [EFD1] -> Mux9/1
  [dtheta2] -> Mux2/2
  [dtheta1] -> Mux2/1
  [Pa1] -> To Workspace/1, Mux1/1, Mux4/1
  Mux9/1 -> Field voltage/1, W8/1
  [Pa3] -> To Workspace11/1, Mux5/1, Mux4/3
  [EFD2] -> Mux9/2
  [Pe3] -> W10/1, Mux8/3
  [pss3] -> Mux7/3
  [Vt4] -> Mux6/4
  Mux6/1 -> Vt/1, Terminal voltage/1, W6/1  "Vt"
  [dtheta4] -> Mux2/4
  [Pe1] -> Scope2/1, W2/1, Mux8/1
  Mux4/1 -> Accelerating power/1, Pa/1, W1/1  "Pa"
  [pss1] -> Mux7/1
  Mux1/1 -> Scope/1, To Workspace6/1  "Pa12"
  Mux5/1 -> To Workspace7/1, Scope1/1  "Pa12"
  [Pe4] -> Scope3/1, W3/1, Mux8/4
  [PB1] -> Mux12/1
  [PB4] -> Mux12/4
  [PB3] -> Mux12/3
  [PB2] -> Mux12/2
  Mux12/1 -> To Workspace8/1, Scope4/1
  [DELTA3] -> Mux14/3
  [DELTA4] -> Mux14/4
  [DELTA2] -> Mux14/2
  [DELTA1] -> Mux14/1
  Mux14/1 -> To Workspace10/1, Scope6/1

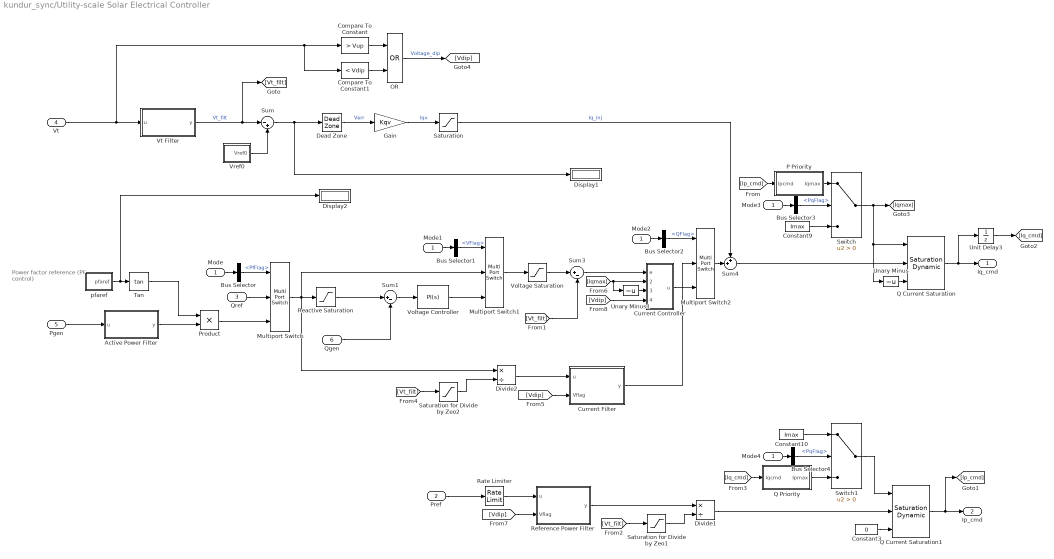
== system kundur_sync/Utility-scale Solar Electrical Controller ==
  note: Power factor reference (PF control)
  Mode : Inport
  Pref : Inport  Port=2
  Qref : Inport  Port=3
  Vt : Inport  Port=4
  Pgen : Inport  Port=5
  Qgen : Inport  Port=6
  Active Power Filter : Subsystem  mask{k=1, tau=Tp, vmax=Inf, vmin=-Inf}
      mask Display: fprintf('1\n------------\n(1 + s Tp)');
  Bus Selector : BusSelector  OutputSignals=PfFlag
  Bus Selector1 : BusSelector  OutputSignals=VFlag
  Bus Selector2 : BusSelector  OutputSignals=QFlag
  Bus Selector3 : BusSelector  OutputSignals=PqFlag
  Bus Selector4 : BusSelector  OutputSignals=PqFlag
  Compare To Constant : simulink/Logic and Bit Operations/Compare To Constant  relop=>  const=Vup  OutDataTypeStr=boolean
  Compare To Constant1 : simulink/Logic and Bit Operations/Compare To Constant  relop=<  const=Vdip  OutDataTypeStr=boolean
  Constant10 : Constant  Value=Imax
  Constant3 : Constant  Value=0
  Constant9 : Constant  Value=Imax
  Current Controller : Subsystem
  Current Filter : Subsystem  mask{k=1, tau=Tiq, vmax=Inf, vmin=-Inf}
      mask Display: fprintf('1\n------------\n(1 + s Tiq)');
  Dead Zone : DeadZone  LowerValue=dbd1  UpperValue=dbd2
  Display1 : Display
  Display2 : Display
  Divide1 : Product  Inputs=*/
  Divide2 : Product  Inputs=*/
  Gain : Gain  Gain=Kqv
  Mode{1..4} (4 alike) : InportShadow
  Multiport Switch : MultiPortSwitch  DataPortOrder=Zero-based contiguous  Inputs=2  zeroidx=on  SaturateOnIntegerOverflow=off  InputSameDT=off
  Multiport Switch1 : MultiPortSwitch  DataPortOrder=Zero-based contiguous  Inputs=2  zeroidx=on  SaturateOnIntegerOverflow=off  InputSameDT=off
  Multiport Switch2 : MultiPortSwitch  DataPortOrder=Zero-based contiguous  Inputs=2  zeroidx=on  SaturateOnIntegerOverflow=off  InputSameDT=off
  OR : Logic  Operator=OR  AllPortsSameDT=off  OutDataTypeStr=boolean
  P Priority : Subsystem
  Product : Product
  Q Current Saturation : simulink/Discontinuities/Saturation Dynamic  OutMin=[]  OutMax=[]  OutDataTypeStr=Inherit: Same as second input  OutDataType=fixdt(1, 16)  OutScaling=2^-10  DoSatur=off
  Q Current Saturation1 : simulink/Discontinuities/Saturation Dynamic  OutMin=[]  OutMax=[]  OutDataTypeStr=Inherit: Same as second input  OutDataType=fixdt(1, 16)  OutScaling=2^-10  DoSatur=off
  Q Priority : Subsystem
  Rate Limiter : RateLimiter  RisingSlewLimit=dPmax  FallingSlewLimit=dPmin  SampleTimeMode=inherited
  Reactive Saturation : Saturate  UpperLimit=Qmax  LowerLimit=Qmin
  Reference Power Filter : Subsystem  mask{k=1, tau=Tpord, vmax=Pmax, vmin=Pmin}
      mask Display: fprintf('1\n------------\n(1 + s Tpord)');
  Saturation : Saturate  UpperLimit=Iqhl  LowerLimit=Iqll
  Saturation for Divide by Zeo1 : Saturate  UpperLimit=inf  LowerLimit=0.01
  Saturation for Divide by Zeo2 : Saturate  UpperLimit=inf  LowerLimit=0.01
  Sum : Sum  Inputs=|-+
  Sum1 : Sum  Inputs=|+-
  Sum3 : Sum  Inputs=|+-
  Sum4 : Sum  Inputs=++|
  Switch : Switch  Criteria=u2 > Threshold  SaturateOnIntegerOverflow=off  InputSameDT=off
  Switch1 : Switch  Criteria=u2 > Threshold  SaturateOnIntegerOverflow=off  InputSameDT=off
  Tan : Trigonometry  Operator=tan
  Unary Minus : UnaryMinus
  Unary Minus1 : UnaryMinus
  Unit Delay3 : UnitDelay  SampleTime=-1  HasFrameUpgradeWarning=on
  Voltage Controller : slpidlib/PID Controller  Controller=PI  Form=Parallel  TimeDomain=Continuous-time  UseExternalTs=off  SampleTime=-1  IntegratorMethod=Forward Euler  FilterMethod=Forward Euler  ControllerParametersSource=internal  P=Kqp  I=Kqi  UseKiTs=off  D=0  N=100  UseFilter=on  TunerSelectOption=Transfer Function Based (PID Tuner App)  InitialConditionSource=internal  InitialConditionForIntegrator=1  InitialConditionForFilter=0  DifferentiatorICPrevScaledInput=0  ExternalReset=none  TrackingMode=off  Kt=1  LimitOutput=on  SatLimitsSource=internal  UpperSaturationLimit=Vmax  LowerSaturationLimit=Vmin  LinearizeAsGain=on  AntiWindupMode=none  Kb=1  LimitIntegrator=off  UpperIntegratorSaturationLimit=inf  LowerIntegratorSaturationLimit=-inf  POutMin=[]  POutMax=[]  IOutMin=[]  IOutMax=[]  DOutMin=[]  DOutMax=[]  NOutMin=[]  NOutMax=[]  SumOutMin=[]  SumOutMax=[]  SaturationOutMin=[]  SaturationOutMax=[]  PParamMin=[]  PParamMax=[]  IParamMin=[]  IParamMax=[]  DParamMin=[]  DParamMax=[]  NParamMin=[]  NParamMax=[]  KbParamMin=[]  KbParamMax=[]  KtParamMin=[]  KtParamMax=[]  KbOutMin=[]  KbOutMax=[]  KtOutMin=[]  KtOutMax=[]  IntegratorOutMin=[]  IntegratorOutMax=[]  FilterOutMin=[]  FilterOutMax=[]  SumI1OutMin=[]  SumI1OutMax=[]  SumI2OutMin=[]  SumI2OutMax=[]  SumI3OutMin=[]  SumI3OutMax=[]  SumI4OutMin=[]  SumI4OutMax=[]  SumDOutMin=[]  SumDOutMax=[]  DifferentiatorOutMin=[]  DifferentiatorOutMax=[]  FilterDiffOutCoefMin=[]  FilterDiffOutCoefMax=[]  ReciprocalOutMin=[]  ReciprocalOutMax=[]  SumDenOutMin=[]  SumDenOutMax=[]  SumNumOutMin=[]  SumNumOutMax=[]  DivideOutMin=[]  DivideOutMax=[]  UdiffTsProdOutMin=[]  UdiffTsProdOutMax=[]  NTsProdOutMin=[]  NTsProdOutMax=[]  UintegralTsProdOutMin=[]  UintegralTsProdOutMax=[]  UngainTsProdOutMin=[]  UngainTsProdOutMax=[]  ClampingZeroOutDataTypeStr=Inherit: Inherit via back propagation  ClampingZeroOutMin=[]  ClampingZeroOutMax=[]  FilterDenConstantOutDataTypeStr=Inherit: Inherit via back propagation  FilterDenConstantOutMin=[]  FilterDenConstantOutMax=[]  PCopyOutDataTypeStr=Inherit: Inherit via back propagation  PCopyOutMin=[]  PCopyOutMax=[]  NCopyOutDataTypeStr=Inherit: Inherit via back propagation  NCopyOutMin=[]  NCopyOutMax=[]  IntegratorContinuousStateAttributes=''  IntegratorStateMustResolveToSignalObject=off  IntegratorRTWStateStorageClass=Auto  FilterContinuousStateAttributes=''  FilterStateMustResolveToSignalObject=off  FilterRTWStateStorageClass=Auto  ParallelPVariant=InternalParameters  IdealPVariant=Disabled  IVariant=InternalParameters  DVariant=Disabled  IntegratorVariant=Continuous  SatVariant=Enabled  AWVariant=Passthrough  PCopyVariant=Disabled  TRVariant=Disabled  FdbkBlocksVariant=Forward  IdealPFdbkVariant=Disabled  SatFdbkVariant=Disabled  DerivativeFilterVariant=Disabled  NVariant=Disabled  NCopyVariant=Disabled_SignalSpec  FilterICVariant=Disabled  IntegratorICVariant=InternalICs  ExternalResetVariant=Disabled  TRSumVariant=Passthrough  SumFdbkVariant=Disabled  SumVariant=Sum_PI  TsampFilterVariant=InternalTs  TsampNgainVariant=Passthrough  TsampIntegralVariant=Disabled_SignalSpec  ExternalSaturationOutDataTypeStr=Inherit: Same as second input
  Voltage Saturation : Saturate  UpperLimit=Vmax  LowerLimit=Vmin
  Vref0 : Subsystem
  Vt Filter : Subsystem  mask{k=1, tau=Trv, vmax=Inf, vmin=-Inf}
      mask Display: fprintf('1\n------------\n(1 + s Trv)');
  pfaref : Subsystem
  Iq_cmd : Outport  VectorParamsAs1DForOutWhenUnconnected=off
  Ip_cmd : Outport  Port=2  VectorParamsAs1DForOutWhenUnconnected=off
  wires:
  Unit Delay3/1 -> [Iq_cmd]
  Qgen/1 -> Sum1/2
  Pgen/1 -> Active Power Filter/1(u)
  Vt/1 -> Vt Filter/1(u), Compare To Constant/1, Compare To Constant1/1
  Vref0/1(Vref0) -> Sum/2
  Reactive Saturation/1 -> Sum1/1
  Voltage Controller/1 -> Multiport Switch1/3
  Bus Selector4/1 -> Switch1/2  "<PqFlag>"
  Sum/1 -> Display1/1, Dead Zone/1
  Multiport Switch/1 -> Reactive Saturation/1, Multiport Switch1/2, Divide2/1
  Voltage Saturation/1 -> Sum3/1
  Bus Selector2/1 -> Multiport Switch2/1  "<QFlag>"
  Vt Filter/1(y) -> Sum/1, [Vt_filt]  "Vt_filt"
  [Iqmax] -> Current Controller/2(umax), Unary Minus1/1
  Constant10/1 -> Switch1/1
  [Vt_filt] -> Sum3/2
  Dead Zone/1 -> Gain/1  "Verr"
  Tan/1 -> Product/1
  Sum3/1 -> Current Controller/1(e)
  Product/1 -> Multiport Switch/3
  Current Controller/1(u) -> Multiport Switch2/3
  Rate Limiter/1 -> Reference Power Filter/1(u)
  Q Current Saturation/1 -> Unit Delay3/1, Iq_cmd/1
  [Vt_filt] -> Saturation for Divide by Zeo1/1
  Current Filter/1(y) -> Multiport Switch2/2
  Sum4/1 -> Q Current Saturation/2
  Unary Minus/1 -> Q Current Saturation/3
  Multiport Switch2/1 -> Sum4/2
  Saturation for Divide by Zeo2/1 -> Divide2/2
  Pref/1 -> Rate Limiter/1
  Multiport Switch1/1 -> Voltage Saturation/1
  Divide1/1 -> Q Current Saturation1/2
  Divide2/1 -> Current Filter/1(u)
  Saturation for Divide by Zeo1/1 -> Divide1/2
  [Ip_cmd] -> P Priority/1(Ipcmd)
  Reference Power Filter/1(y) -> Divide1/1
  pfaref/1(pfaref) -> Display2/1, Tan/1
  OR/1 -> [Vdip]  "Voltage_dip"
  Saturation/1 -> Sum4/1  "Iq_inj"
  Qref/1 -> Multiport Switch/2
  Compare To Constant/1 -> OR/1
  [Vt_filt] -> Saturation for Divide by Zeo2/1
  Bus Selector1/1 -> Multiport Switch1/1  "<VFlag>"
  [Iq_cmd] -> Q Priority/1(Iqcmd)
  Q Priority/1(Ipmax) -> Switch1/3
  Gain/1 -> Saturation/1  "Iqv"
  Switch1/1 -> Q Current Saturation1/1
  Sum1/1 -> Voltage Controller/1
  Constant3/1 -> Q Current Saturation1/3
  Switch/1 -> Unary Minus/1, Q Current Saturation/1, [Iqmax]
  Compare To Constant1/1 -> OR/2
  Active Power Filter/1(y) -> Product/2
  P Priority/1(Iqmax) -> Switch/1
  Constant9/1 -> Switch/3
  Q Current Saturation1/1 -> Ip_cmd/1, [Ip_cmd]
  [Vdip] -> Reference Power Filter/2(Vflag)
  [Vdip] -> Current Filter/2(Vflag)
  [Vdip] -> Current Controller/4(Vdip)
  Unary Minus1/1 -> Current Controller/3(umin)
  Mode/1 -> Bus Selector/1
  Bus Selector/1 -> Multiport Switch/1  "<PfFlag>"
  Mode1/1 -> Bus Selector1/1
  Mode2/1 -> Bus Selector2/1
  Mode3/1 -> Bus Selector3/1
  Bus Selector3/1 -> Switch/2  "<PqFlag>"
  Mode4/1 -> Bus Selector4/1

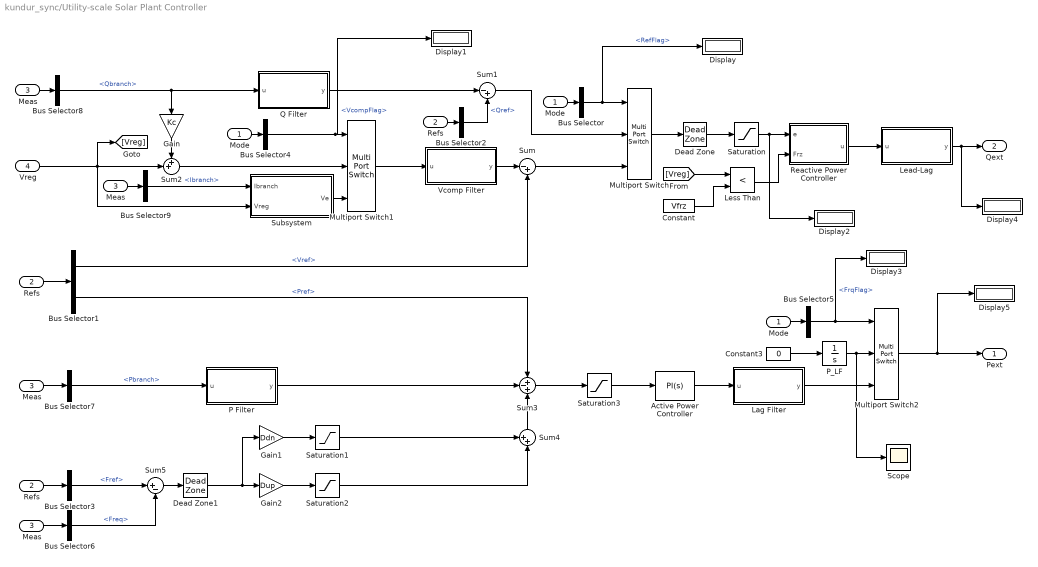
== system kundur_sync/Utility-scale Solar Plant Controller ==
  Mode : Inport
  Refs : Inport  Port=2
  " Meas" : Inport  Port=3
  Vreg : Inport  Port=4
  "  Meas" : InportShadow  Port=3
  "  Meas " : InportShadow  Port=3
  " Meas " : InportShadow  Port=3
  " Mode" : InportShadow
  " Refs" : InportShadow  Port=2
  Active Power Controller : slpidlib/PID Controller  Controller=PI  Form=Parallel  TimeDomain=Continuous-time  UseExternalTs=off  SampleTime=-1  IntegratorMethod=Forward Euler  FilterMethod=Forward Euler  ControllerParametersSource=internal  P=Kpg  I=Kig  UseKiTs=off  D=0  N=100  UseFilter=on  TunerSelectOption=Transfer Function Based (PID Tuner App)  InitialConditionSource=internal  InitialConditionForIntegrator=1  InitialConditionForFilter=0  DifferentiatorICPrevScaledInput=0  ExternalReset=none  TrackingMode=off  Kt=1  LimitOutput=on  SatLimitsSource=internal  UpperSaturationLimit=Pmax  LowerSaturationLimit=Pmin  LinearizeAsGain=on  AntiWindupMode=none  Kb=1  LimitIntegrator=off  UpperIntegratorSaturationLimit=inf  LowerIntegratorSaturationLimit=-inf  POutMin=[]  POutMax=[]  IOutMin=[]  IOutMax=[]  DOutMin=[]  DOutMax=[]  NOutMin=[]  NOutMax=[]  SumOutMin=[]  SumOutMax=[]  SaturationOutMin=[]  SaturationOutMax=[]  PParamMin=[]  PParamMax=[]  IParamMin=[]  IParamMax=[]  DParamMin=[]  DParamMax=[]  NParamMin=[]  NParamMax=[]  KbParamMin=[]  KbParamMax=[]  KtParamMin=[]  KtParamMax=[]  KbOutMin=[]  KbOutMax=[]  KtOutMin=[]  KtOutMax=[]  IntegratorOutMin=[]  IntegratorOutMax=[]  FilterOutMin=[]  FilterOutMax=[]  SumI1OutMin=[]  SumI1OutMax=[]  SumI2OutMin=[]  SumI2OutMax=[]  SumI3OutMin=[]  SumI3OutMax=[]  SumI4OutMin=[]  SumI4OutMax=[]  SumDOutMin=[]  SumDOutMax=[]  DifferentiatorOutMin=[]  DifferentiatorOutMax=[]  FilterDiffOutCoefMin=[]  FilterDiffOutCoefMax=[]  ReciprocalOutMin=[]  ReciprocalOutMax=[]  SumDenOutMin=[]  SumDenOutMax=[]  SumNumOutMin=[]  SumNumOutMax=[]  DivideOutMin=[]  DivideOutMax=[]  UdiffTsProdOutMin=[]  UdiffTsProdOutMax=[]  NTsProdOutMin=[]  NTsProdOutMax=[]  UintegralTsProdOutMin=[]  UintegralTsProdOutMax=[]  UngainTsProdOutMin=[]  UngainTsProdOutMax=[]  ClampingZeroOutDataTypeStr=Inherit: Inherit via back propagation  ClampingZeroOutMin=[]  ClampingZeroOutMax=[]  FilterDenConstantOutDataTypeStr=Inherit: Inherit via back propagation  FilterDenConstantOutMin=[]  FilterDenConstantOutMax=[]  PCopyOutDataTypeStr=Inherit: Inherit via back propagation  PCopyOutMin=[]  PCopyOutMax=[]  NCopyOutDataTypeStr=Inherit: Inherit via back propagation  NCopyOutMin=[]  NCopyOutMax=[]  IntegratorContinuousStateAttributes=''  IntegratorStateMustResolveToSignalObject=off  IntegratorRTWStateStorageClass=Auto  FilterContinuousStateAttributes=''  FilterStateMustResolveToSignalObject=off  FilterRTWStateStorageClass=Auto  ParallelPVariant=InternalParameters  IdealPVariant=Disabled  IVariant=InternalParameters  DVariant=Disabled  IntegratorVariant=Continuous  SatVariant=Enabled  AWVariant=Passthrough  PCopyVariant=Disabled  TRVariant=Disabled  FdbkBlocksVariant=Forward  IdealPFdbkVariant=Disabled  SatFdbkVariant=Disabled  DerivativeFilterVariant=Disabled  NVariant=Disabled  NCopyVariant=Disabled_SignalSpec  FilterICVariant=Disabled  IntegratorICVariant=InternalICs  ExternalResetVariant=Disabled  TRSumVariant=Passthrough  SumFdbkVariant=Disabled  SumVariant=Sum_PI  TsampFilterVariant=InternalTs  TsampNgainVariant=Passthrough  TsampIntegralVariant=Disabled_SignalSpec  ExternalSaturationOutDataTypeStr=Inherit: Same as second input
  Bus Selector : BusSelector  OutputSignals=RefFlag
  Bus Selector1 : BusSelector  OutputSignals=Vref,Pref
  Bus Selector2 : BusSelector  OutputSignals=Qref
  Bus Selector3 : BusSelector  OutputSignals=Fref
  Bus Selector4 : BusSelector  OutputSignals=VcompFlag
  Bus Selector5 : BusSelector  OutputSignals=FrqFlag
  Bus Selector6 : BusSelector  OutputSignals=Freq
  Bus Selector7 : BusSelector  OutputSignals=Pbranch
  Bus Selector8 : BusSelector  OutputSignals=Qbranch
  Bus Selector9 : BusSelector  OutputSignals=Ibranch
  Constant : Constant  Value=Vfrz
  Constant3 : Constant  Value=0
  Dead Zone : DeadZone  LowerValue=-db1  UpperValue=db1
  Dead Zone1 : DeadZone  LowerValue=fdbd1  UpperValue=fdbd2
  Display{,1..5} (6 alike) : Display
  Gain : Gain  Gain=Kc
  Gain1 : Gain  Gain=Ddn
  Gain2 : Gain  Gain=Dup
  Lag Filter : Subsystem  mask{k=1, tau=Tlag, vmax=Inf, vmin=-Inf}
      mask Display: fprintf('1\n------------\n(1 + s Tlag)');
  Lead-Lag : Subsystem  mask{ta=Tft, tb=Tfv}
      mask prompts: ta "numerator tau (ta)"; tb "denominator tau  (tb)"
      mask Display: fprintf('(1 + s Tft)\n------------\n(1 + s Tfv)');
  Less Than : RelationalOperator  Operator=<  OutDataTypeStr=boolean  RndMeth=Simplest  InputSameDT=off
  "Mode " : InportShadow
  Multiport Switch : MultiPortSwitch  DataPortOrder=Zero-based contiguous  Inputs=2  zeroidx=on  SaturateOnIntegerOverflow=off  InputSameDT=off
  Multiport Switch1 : MultiPortSwitch  DataPortOrder=Zero-based contiguous  Inputs=2  zeroidx=on  SaturateOnIntegerOverflow=off  InputSameDT=off
  Multiport Switch2 : MultiPortSwitch  DataPortOrder=Zero-based contiguous  Inputs=2  zeroidx=on  SaturateOnIntegerOverflow=off  InputSameDT=off
  P Filter : Subsystem  mask{k=1, tau=Tp, vmax=Inf, vmin=-Inf}
      mask Display: fprintf('1\n------------\n(1 + s Tfltr)');
  P_LF : Integrator  InitialCondition=1
  Q Filter : Subsystem  mask{k=1, tau=Tfltr, vmax=Inf, vmin=-Inf}
      mask Display: fprintf('1\n------------\n(1 + s Tfltr)');
  Reactive Power Controller : Subsystem
  "Refs " : InportShadow  Port=2
  Saturation : Saturate  UpperLimit=emax  LowerLimit=emin
  Saturation1 : Saturate  UpperLimit=0  LowerLimit=-inf
  Saturation2 : Saturate  UpperLimit=inf  LowerLimit=0
  Saturation3 : Saturate  UpperLimit=femax  LowerLimit=femin
  Scope : Scope
  Subsystem : Subsystem
  Sum : Sum  Inputs=|-+
  Sum1 : Sum  Inputs=|-+
  Sum2 : Sum  Inputs=++|
  Sum3 : Sum  Inputs=+-+
  Sum4 : Sum  Inputs=++|
  Sum5 : Sum  Inputs=|+-
  Vcomp Filter : Subsystem  mask{k=1, tau=Tfltr, vmax=Inf, vmin=-Inf}
      mask Display: fprintf('1\n------------\n(1 + s Tfltr)');
  Pext : Outport  VectorParamsAs1DForOutWhenUnconnected=off
  Qext : Outport  Port=2  VectorParamsAs1DForOutWhenUnconnected=off
  wires:
  Vreg/1 -> [Vreg], Sum2/2, Subsystem/2(Vreg)
  "  Meas "/1 -> Bus Selector9/1
  "  Meas"/1 -> Bus Selector8/1
  " Meas "/1 -> Bus Selector7/1
  " Meas"/1 -> Bus Selector6/1
  " Mode"/1 -> Bus Selector5/1
  Bus Selector4/1 -> Display1/1, Multiport Switch1/1  "<VcompFlag>"
  "Mode "/1 -> Bus Selector4/1
  " Refs"/1 -> Bus Selector3/1
  "Refs "/1 -> Bus Selector2/1
  Refs/1 -> Bus Selector1/1
  Mode/1 -> Bus Selector/1
  Bus Selector1/1 -> Sum/2  "<Vref>"
  Gain/1 -> Sum2/1
  P Filter/1(y) -> Sum3/2
  Bus Selector6/1 -> Sum5/2  "<Freq>"
  Bus Selector8/1 -> Q Filter/1(u), Gain/1  "<Qbranch>"
  Bus Selector3/1 -> Sum5/1  "<Fref>"
  Multiport Switch1/1 -> Vcomp Filter/1(u)
  Sum2/1 -> Multiport Switch1/2
  Vcomp Filter/1(y) -> Sum/1
  Reactive Power Controller/1(u) -> Lead-Lag/1(u)
  Bus Selector2/1 -> Sum1/2  "<Qref>"
  Lead-Lag/1(y) -> Display4/1, Qext/1
  Subsystem/1(Ve) -> Multiport Switch1/3
  Bus Selector1/2 -> Sum3/1  "<Pref>"
  Bus Selector7/1 -> P Filter/1(u)  "<Pbranch>"
  Gain2/1 -> Saturation2/1
  Saturation2/1 -> Sum4/2
  Active Power Controller/1 -> Lag Filter/1(u)
  Lag Filter/1(y) -> Multiport Switch2/3
  Bus Selector5/1 -> Display3/1, Multiport Switch2/1  "<FrqFlag>"
  Dead Zone1/1 -> Gain2/1, Gain1/1
  Multiport Switch2/1 -> Display5/1, Pext/1
  Multiport Switch/1 -> Dead Zone/1
  Gain1/1 -> Saturation1/1
  Sum3/1 -> Saturation3/1
  Bus Selector9/1 -> Subsystem/1(Ibranch)  "<Ibranch>"
  Bus Selector/1 -> Display/1, Multiport Switch/1  "<RefFlag>"
  Saturation/1 -> Display2/1, Reactive Power Controller/1(e)
  Sum5/1 -> Dead Zone1/1
  Saturation1/1 -> Sum4/1
  Sum1/1 -> Multiport Switch/2
  Sum4/1 -> Sum3/3
  Q Filter/1(y) -> Sum1/1
  Saturation3/1 -> Active Power Controller/1
  Dead Zone/1 -> Saturation/1
  Constant3/1 -> P_LF/1
  Sum/1 -> Multiport Switch/3
  [Vreg] -> Less Than/1
  Less Than/1 -> Reactive Power Controller/2(Frz)
  Constant/1 -> Less Than/2
  P_LF/1 -> Scope/1, Multiport Switch2/2

== system kundur_sync/Renewable Grid-Connection/Break F Loop ==
  u : Inport
  Gain2 : Gain  Gain=1/tau
  Integrator2 : Integrator  InitialCondition=1
  Sum3 : Sum  Inputs=|+-
  to PU1 : Gain  Gain=toPU
  to PU7 : Gain  Gain=1/toPU
  y : Outport  VectorParamsAs1DForOutWhenUnconnected=off
  wires:
  to PU1/1 -> y/1
  to PU7/1 -> Sum3/1
  u/1 -> to PU7/1
  Sum3/1 -> Gain2/1
  Integrator2/1 -> Sum3/2, to PU1/1
  Gain2/1 -> Integrator2/1
